simulink model "scheme_L2"  (R2026b)
settings: Solver=VariableStepAuto  StopTime=10  MaxStep=0.01
settings Model: Creator=Anna  LastModifiedBy=Anna

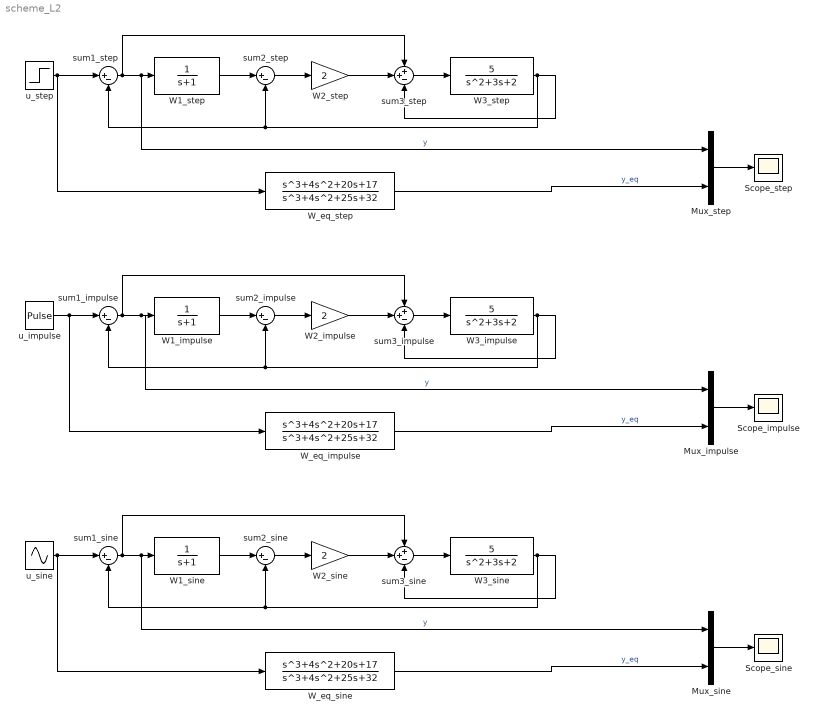
== system scheme_L2 ==
  Mux_impulse : Mux  Inputs=2
  Mux_sine : Mux  Inputs=2
  Mux_step : Mux  Inputs=2
  Scope_impulse : Scope
  Scope_sine : Scope
  Scope_step : Scope
      settings: ActiveDisplayYMinimum=-0.12499999999999997  ActiveDisplayYMaximum=1.125
  W1_impulse : TransferFcn  Numerator=1  Denominator=[1 1]
  W1_sine : TransferFcn  Numerator=1  Denominator=[1 1]
  W1_step : TransferFcn  Numerator=1  Denominator=[1 1]
  W2_impulse : Gain  Gain=2
  W2_sine : Gain  Gain=2
  W2_step : Gain  Gain=2
  W3_impulse : TransferFcn  Numerator=5  Denominator=[1 3 2]
  W3_sine : TransferFcn  Numerator=5  Denominator=[1 3 2]
  W3_step : TransferFcn  Numerator=5  Denominator=[1 3 2]
  W_eq_impulse : TransferFcn  Numerator=[1 4 20 17]  Denominator=[1 4 25 32]
  W_eq_sine : TransferFcn  Numerator=[1 4 20 17]  Denominator=[1 4 25 32]
  W_eq_step : TransferFcn  Numerator=[1 4 20 17]  Denominator=[1 4 25 32]
  sum1_impulse : Sum  Inputs=|+-
  sum1_sine : Sum  Inputs=|+-
  sum1_step : Sum  Inputs=|+-
  sum2_impulse : Sum  Inputs=|+-
  sum2_sine : Sum  Inputs=|+-
  sum2_step : Sum  Inputs=|+-
  sum3_impulse : Sum  Inputs=++-
  sum3_sine : Sum  Inputs=++-
  sum3_step : Sum  Inputs=++-
  u_impulse : DiscretePulseGenerator  PulseType=Time based  Amplitude=10  Period=10  PhaseDelay=1
  u_sine : Sin  SampleTime=0
  u_step : Step  SampleTime=0
  wires:
  u_step/1 -> sum1_step/1, W_eq_step/1
  sum1_step/1 -> W1_step/1, Mux_step/1, sum3_step/1  "y"
  W1_step/1 -> sum2_step/1
  sum2_step/1 -> W2_step/1
  W2_step/1 -> sum3_step/2
  sum3_step/1 -> W3_step/1
  W3_step/1 -> sum2_step/2, sum1_step/2, sum3_step/3
  W_eq_step/1 -> Mux_step/2  "y_eq"
  Mux_step/1 -> Scope_step/1
  u_impulse/1 -> sum1_impulse/1, W_eq_impulse/1
  sum1_impulse/1 -> W1_impulse/1, Mux_impulse/1, sum3_impulse/1  "y"
  W1_impulse/1 -> sum2_impulse/1
  sum2_impulse/1 -> W2_impulse/1
  W2_impulse/1 -> sum3_impulse/2
  sum3_impulse/1 -> W3_impulse/1
  W3_impulse/1 -> sum2_impulse/2, sum1_impulse/2, sum3_impulse/3
  W_eq_impulse/1 -> Mux_impulse/2  "y_eq"
  Mux_impulse/1 -> Scope_impulse/1
  u_sine/1 -> sum1_sine/1, W_eq_sine/1
  sum1_sine/1 -> W1_sine/1, Mux_sine/1, sum3_sine/1  "y"
  W1_sine/1 -> sum2_sine/1
  sum2_sine/1 -> W2_sine/1
  W2_sine/1 -> sum3_sine/2
  sum3_sine/1 -> W3_sine/1
  W3_sine/1 -> sum2_sine/2, sum1_sine/2, sum3_sine/3
  W_eq_sine/1 -> Mux_sine/2  "y_eq"
  Mux_sine/1 -> Scope_sine/1
